simulink model "hrg_periodic_shared"  (R2025a)
settings: Solver=FixedStepDiscrete  StartTime=0.0  StopTime=c.duration  FixedStep=c.Ts  RelTol=1e-3
model workspace (MAT data in the model file):
  c : object (value not decoded)
symbols that are objects in the model workspace (value not decoded): c
(part 2 of 2)

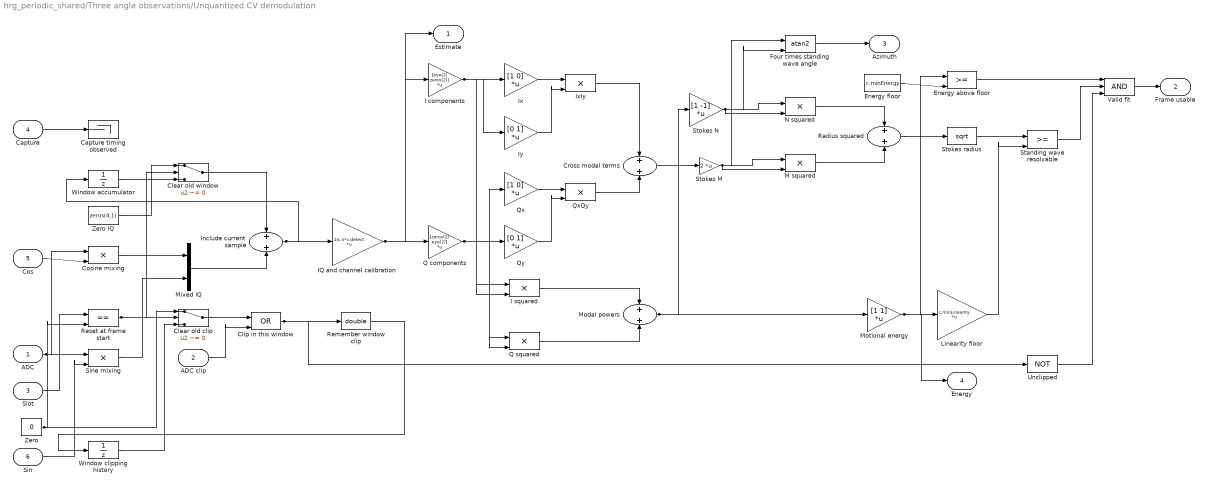
== system hrg_periodic_shared/Three angle observations/Unquantized CV demodulation ==
  ADC : Inport
  ADC clip : Inport  Port=2
  Slot : Inport  Port=3
  Capture : Inport  Port=4
  Cos : Inport  Port=5
  Sin : Inport  Port=6
  Capture timing observed : Terminator
  Clear old clip : Switch  Criteria=u2 ~= 0  SaturateOnIntegerOverflow=off  InputSameDT=off
  Clear old window : Switch  Criteria=u2 ~= 0  SaturateOnIntegerOverflow=off  InputSameDT=off
  Clip in this window : Logic  Operator=OR  AllPortsSameDT=off  OutDataTypeStr=boolean
  Cosine mixing : Product
  Cross modal terms : Sum
  Energy above floor : RelationalOperator  OutDataTypeStr=boolean  RndMeth=Simplest  InputSameDT=off
  Energy floor : Constant  Value=c.minEnergy
  Four times standing wave angle : Trigonometry  Operator=atan2
  I components : Gain  Gain=[eye(2) zeros(2)]  Multiplication=Matrix(K*u)
  I squared : Product
  IQ and channel calibration : Gain  Gain=2/c.n*c.detect  Multiplication=Matrix(K*u)
  Include current sample : Sum
  Ix : Gain  Gain=[1 0]  Multiplication=Matrix(K*u)
  IxIy : Product
  Iy : Gain  Gain=[0 1]  Multiplication=Matrix(K*u)
  Linearity floor : Gain  Gain=c.minLinearity  Multiplication=Matrix(K*u)
  M squared : Product
  Mixed IQ : Mux  Inputs=2
  Modal powers : Sum
  Motional energy : Gain  Gain=[1 1]  Multiplication=Matrix(K*u)
  N squared : Product
  Q components : Gain  Gain=[zeros(2) eye(2)]  Multiplication=Matrix(K*u)
  Q squared : Product
  Qx : Gain  Gain=[1 0]  Multiplication=Matrix(K*u)
  QxQy : Product
  Qy : Gain  Gain=[0 1]  Multiplication=Matrix(K*u)
  Radius squared : Sum
  Remember window clip : DataTypeConversion  OutDataTypeStr=double  SaturateOnIntegerOverflow=off  RndMeth=Floor
  Reset at frame start : RelationalOperator  Operator===  OutDataTypeStr=boolean  RndMeth=Simplest  InputSameDT=off
  Sine mixing : Product
  Standing wave resolvable : RelationalOperator  OutDataTypeStr=boolean  RndMeth=Simplest  InputSameDT=off
  Stokes M : Gain  Gain=2  Multiplication=Matrix(K*u)
  Stokes N : Gain  Gain=[1 -1]  Multiplication=Matrix(K*u)
  Stokes radius : Sqrt
  Unclipped : Logic  Operator=NOT  Inputs=1  AllPortsSameDT=off  OutDataTypeStr=boolean
  Valid fit : Logic  Inputs=3  AllPortsSameDT=off  OutDataTypeStr=boolean
  Window accumulator : UnitDelay  InitialCondition=zeros(4,1)  SampleTime=c.Ts  HasFrameUpgradeWarning=on
  Window clipping history : UnitDelay  SampleTime=c.Ts  HasFrameUpgradeWarning=on
  Zero : Constant  Value=0
  Zero IQ : Constant  Value=zeros(4,1)
  Estimate : Outport
  Frame usable : Outport  Port=2
  Azimuth : Outport  Port=3
  Energy : Outport  Port=4
  wires:
  Clip in this window/1 -> Unclipped/1, Remember window clip/1
  Zero IQ/1 -> Clear old window/1
  Radius squared/1 -> Stokes radius/1
  Zero/1 -> Clear old clip/1, Reset at frame start/2
  Energy floor/1 -> Energy above floor/2
  ADC/1 -> Cosine mixing/1, Sine mixing/1
  Stokes N/1 -> Four times standing wave angle/2, N squared/1, N squared/2
  Capture/1 -> Capture timing observed/1
  QxQy/1 -> Cross modal terms/2
  Cos/1 -> Cosine mixing/2
  ADC clip/1 -> Clip in this window/2
  Sin/1 -> Sine mixing/2
  Slot/1 -> Reset at frame start/1
  Window accumulator/1 -> Clear old window/3
  Cosine mixing/1 -> Mixed IQ/1
  Iy/1 -> IxIy/2
  Reset at frame start/1 -> Clear old window/2, Clear old clip/2
  Sine mixing/1 -> Mixed IQ/2
  Window clipping history/1 -> Clear old clip/3
  Energy above floor/1 -> Valid fit/1
  Clear old window/1 -> Include current sample/1
  Mixed IQ/1 -> Include current sample/2
  Clear old clip/1 -> Clip in this window/1
  Motional energy/1 -> Energy above floor/1, Linearity floor/1, Energy/1
  Include current sample/1 -> Window accumulator/1, IQ and channel calibration/1
  IQ and channel calibration/1 -> I components/1, Q components/1, Estimate/1
  Remember window clip/1 -> Window clipping history/1
  I components/1 -> I squared/2, I squared/1, Ix/1, Iy/1
  Q components/1 -> Q squared/2, Qx/1, Qy/1, Q squared/1
  Ix/1 -> IxIy/1
  Qx/1 -> QxQy/1
  Linearity floor/1 -> Standing wave resolvable/2
  I squared/1 -> Modal powers/1
  Qy/1 -> QxQy/2
  Q squared/1 -> Modal powers/2
  IxIy/1 -> Cross modal terms/1
  Cross modal terms/1 -> Stokes M/1
  Modal powers/1 -> Motional energy/1, Stokes N/1
  Stokes M/1 -> Four times standing wave angle/1, M squared/1, M squared/2
  Four times standing wave angle/1 -> Azimuth/1
  N squared/1 -> Radius squared/1
  M squared/1 -> Radius squared/2
  Stokes radius/1 -> Standing wave resolvable/1
  Standing wave resolvable/1 -> Valid fit/2
  Unclipped/1 -> Valid fit/3
  Valid fit/1 -> Frame usable/1

== system hrg_periodic_shared/Trace/Frame records ==
  Data : Inport
  Enable : EnablePort
  Export frames : ToWorkspace  VariableName=frames  SampleTime=-1
  wires:
  Data/1 -> Export frames/1
